simulink model "Lab2_VM_Task_3"  (R2024b)
settings: Solver=FixedStepDiscrete  StartTime=0.0  StopTime=Inf  FixedStep=0.02  RelTol=1e-3  EnableMultiTasking=on
values from neighbouring files (symbols this model uses):
  L = [-a 1 -b]    [make_line_task3.m]    (also in make_traj_task2.m = 5; plot_task1.m = 0.1)
undefined symbols (not defined in the file or in its folder): Angular, Linear
libraries: robotlib x3
settings Model: Creator=The MathWorks, Inc.  LastModifiedBy=david
settings SolverCC: AlgebraicLoopSolver=TrustRegion
settings DataIOCC: LimitDataPoints=on  SaveFormat=Array  ReturnWorkspaceOutputs=off
settings OptimizationCC: ZeroExternalMemoryAtStartup=off  ZeroInternalMemoryAtStartup=off  LifeSpan=Inf  MaxStackSize=64
settings DebuggingCC: SolverPrmCheckMsg=warning  UnconnectedInputMsg=warning  UnconnectedOutputMsg=warning  UnconnectedLineMsg=warning  AllowSymbolicDim=off  SFUnexpectedBacktrackingDiag=warning  SFNoUnconditionalDefaultTransitionDiag=warning  SFExecutionAtInitializationDiag=none  ArithmeticOperatorsInVariantConditions=warning
settings HardwareCC: ProdBitPerPointer=32  ProdBitPerSizeT=32  ProdBitPerPtrDiffT=32  ProdLargestAtomicFloat=None  ProdIntDivRoundTo=Undefined  ProdEndianess=Unspecified  ProdWordSize=32  ProdHWDeviceType=Generic->Unspecified (assume 32-bit Generic)  TargetHWDeviceType=Generic->Unspecified (assume 32-bit Generic)  UseEmbeddedCoderFeatures=off
settings ModelReferenceCC: EnableRefExpFcnMdlSchedulingChecks=on  PropagateSignalLabelsOutOfModel=off
settings SFSimCC: SimUseLocalCustomCode=off  CustomCodeUndefinedFunction=UseInterfaceOnly  SimTargetLang=C++
settings RTWCC: Description=Embedded Coder  SystemTargetFile=ert.tlc  HardwareBoard=Robot Operating System (ROS)  TemplateMakefile=ert_default_tmf  RTWUseLocalCustomCode=off  Toolchain=Catkin  TargetLang=C++  GPUComputeCapability=3.5
settings CodeAppCC: StateflowObjectComments=on
settings ERTTargetCC: MultiwordLength=2048  ERTCustomFileBanners=off  CodeInterfacePackaging=C++ class  SupportContinuousTime=on  SupportNonInlinedSFcns=on  RemoveResetFunc=off  SupportVariableSizeSignals=on  ModelStepFunctionPrototypeControlCompliant=off  InlinedParameterPlacement=Hierarchical  RootIOFormat=Structure reference  ConvertIfToSwitch=off  SuppressUnreachableDefaultCases=off  DynamicArrayContainerType=coder::array
settings ConfigComp: CovMetricSettings=dw  CovSaveCumulativeToWorkspaceVar=on  CovSaveSingleToWorkspaceVar=on  CovExternalEMLEnable=off  CovSFcnEnable=off

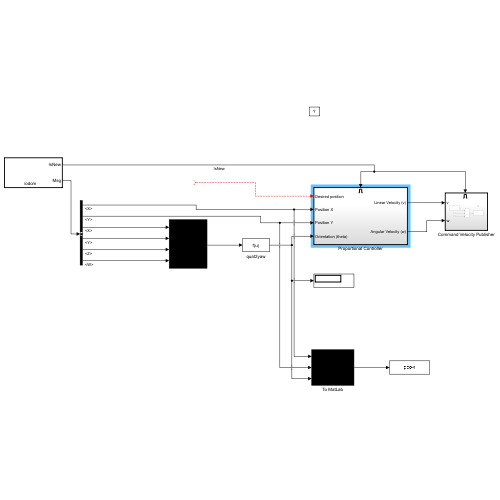
[thumbnail: Simulink's stored preview of the top-level diagram]
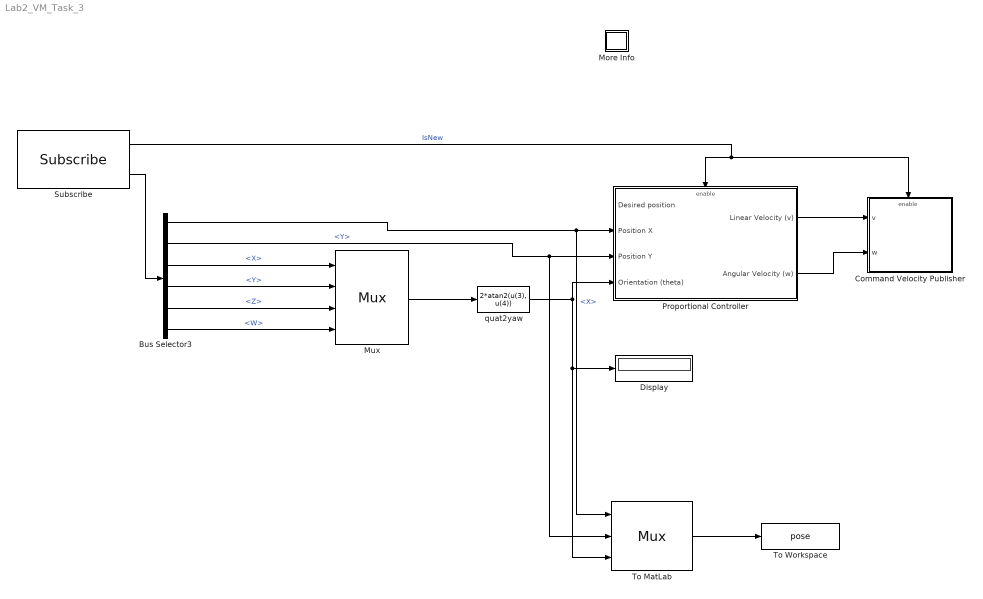
== system Lab2_VM_Task_3 ==
  Bus Selector3 : BusSelector  OutputSignals=Pose.Pose.Position.X,Pose.Pose.Position.Y,Pose.Pose.Orientation.X,Pose.Pose.Orientation.Y,Pose.Pose.Orientation.Z,Pose.Pose.Orientation.W
  Command Velocity Publisher : Subsystem
  Display : Display
  More Info : Subsystem
      settings: OpenFcn=showdemo(bdroot(gcb))
      mask Display: disp('?')
  Mux : Mux
  Proportional Controller : Subsystem
  Subscribe : robotlib/Subscribe  topicSource=Select from ROS network  topic=/odom  messageType=nav_msgs/Odometry  SampleTime=-1  legacyBusStruct=off  messageQueueLength=51
  To MatLab : Mux  Inputs=3
  To Workspace : ToWorkspace  VariableName=pose  SaveFormat=Timeseries  SampleTime=-1
  quat2yaw : Fcn  Expr=2*atan2(u(3), u(4))
  wires:
  Subscribe/2 -> Bus Selector3/1
  Proportional Controller/1(Linear Velocity (v)) -> Command Velocity Publisher/1(v)
  Subscribe/1 -> Command Velocity Publisher/Enable, Proportional Controller/Enable  "IsNew"
  Bus Selector3/5 -> Mux/3  "<Z>"
  Bus Selector3/6 -> Mux/4  "<W>"
  Proportional Controller/2(Angular Velocity (w)) -> Command Velocity Publisher/2(w)
  Bus Selector3/3 -> Mux/1  "<X>"
  Bus Selector3/4 -> Mux/2  "<Y>"
  Mux/1 -> quat2yaw/1
  quat2yaw/1 -> Display/1, To MatLab/3, Proportional Controller/4(Orientation (theta))
  Bus Selector3/1 -> To MatLab/1, Proportional Controller/2(Position X)  "<X>"
  Bus Selector3/2 -> To MatLab/2, Proportional Controller/3(Position Y)  "<Y>"
  ? -> Proportional Controller/1(Desired position)
  To MatLab/1 -> To Workspace/1

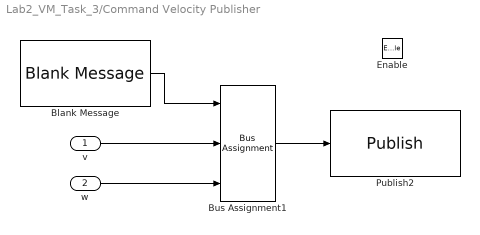
== system Lab2_VM_Task_3/Command Velocity Publisher ==
  v : Inport
  w : Inport  Port=2
  Enable : EnablePort
  Blank Message : robotlib/Blank Message  messageClass=Message  entityType=geometry_msgs/Twist  messageType=geometry_msgs/Twist  SampleTime=inf  legacyBusStruct=off
  Bus Assignment1 : BusAssignment  DialogController=Simulink.DDGSource_BusAssignment  AssignedSignals=Linear.X,Angular.Z
  Publish2 : robotlib/Publish  topicSource=Select from ROS network  topic=/cmd_vel  messageType=geometry_msgs/Twist  legacyBusStruct=off  messageQueueLength=105
  wires:
  Bus Assignment1/1 -> Publish2/1
  Blank Message/1 -> Bus Assignment1/1
  v/1 -> Bus Assignment1/2
  w/1 -> Bus Assignment1/3

== system Lab2_VM_Task_3/More Info ==

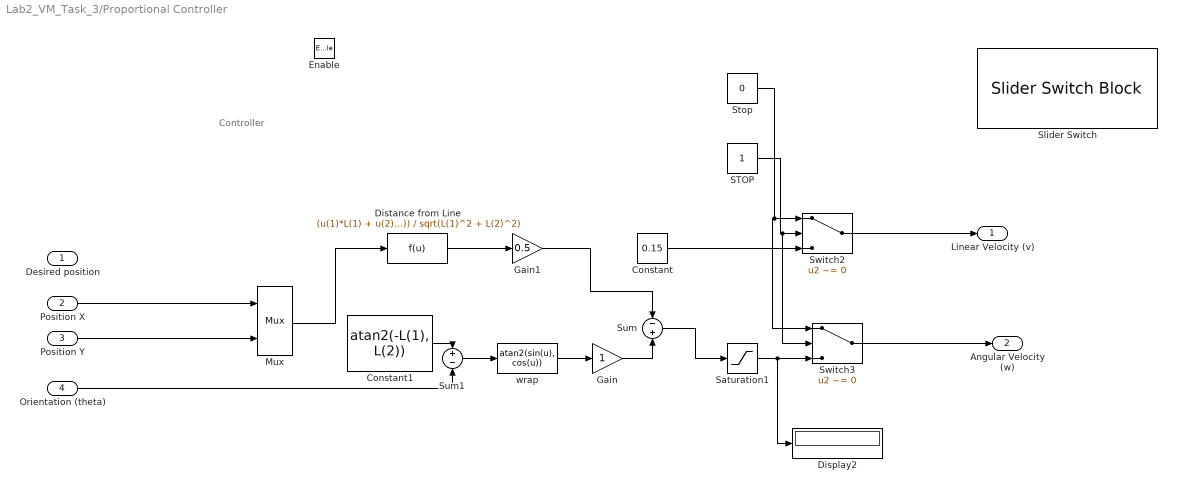
== system Lab2_VM_Task_3/Proportional Controller ==
  note: Controller
  Desired position : Inport
  Position X : Inport  Port=2
  Position Y : Inport  Port=3
  Orientation (theta) : Inport  Port=4
  Enable : EnablePort
  Constant : Constant  Value=0.15
  Constant1 : Constant  Value=atan2(-L(1), L(2))
  Display2 : Display
  Distance from Line : Fcn  Expr=(u(1)*L(1) + u(2)*L(2) + L(3)) / sqrt(L(1)^2 + L(2)^2)
  Gain : Gain
  Gain1 : Gain  Gain=0.5
  Mux : Mux  Inputs=2
  "STOP " : Constant
  Saturation1 : Saturate  UpperLimit=2.84  LowerLimit=-2.84
  Slider Switch : SliderSwitchBlock
      settings: Values={{'Off', 'On'}, [0 1]}
  Stop : Constant  Value=0
  Sum : Sum  Inputs=-+
  Sum1 : Sum  Inputs=+-
  Switch2 : Switch  Criteria=u2 ~= 0  SaturateOnIntegerOverflow=off  InputSameDT=off
  Switch3 : Switch  Criteria=u2 ~= 0  SaturateOnIntegerOverflow=off  InputSameDT=off
  wrap : Fcn  Expr=atan2(sin(u), cos(u))
  Linear Velocity (v) : Outport  VectorParamsAs1DForOutWhenUnconnected=off
  Angular Velocity (w) : Outport  Port=2  VectorParamsAs1DForOutWhenUnconnected=off
  wires:
  Stop/1 -> Switch3/1, Switch2/1
  "STOP "/1 -> Switch3/2, Switch2/2
  Switch2/1 -> Linear Velocity (v)/1
  Switch3/1 -> Angular Velocity (w)/1
  Position X/1 -> Mux/1
  Position Y/1 -> Mux/2
  Orientation (theta)/1 -> Sum1/2
  Sum1/1 -> wrap/1
  wrap/1 -> Gain/1
  Saturation1/1 -> Display2/1, Switch3/3
  Constant/1 -> Switch2/3
  Mux/1 -> Distance from Line/1
  Constant1/1 -> Sum1/1
  Distance from Line/1 -> Gain1/1
  Sum/1 -> Saturation1/1
  Gain1/1 -> Sum/1
  Gain/1 -> Sum/2
